simulink model "FSI09_2"  (R2024b)
settings: Solver=FixedStepAuto  StartTime=0.0  StopTime=t_stop  FixedStep=Ts  RelTol=1e-3
values from neighbouring files (symbols this model uses):
  A = 1+exp(-delta*t)    [FSI04WS.m]    (also in FSI09WS.m = [0 1;-k/m -b/m])
  B = [0;1/m]    [FSI09WS.m]
  C = 0.01    [FSI03WS.m]    (also in FSI09WS.m = [1 0])
  D = [0]    [FSI09WS.m]
  F = 1    [FSI08WS.m]    (also in FSI09WS.m = 10)
  f = chirp_end:(chirp_start/(length(t)-1)):chirp_start    [FSI04WS.m]    (also in FSI08WS.m = 5; FSI09WS.m = 5)
  swich = -1    [FSI08WS.m]    (also in FSI09WS.m; FSI10WS.m)
  t_stop = 500    [FSI04WS.m]    (also in FSI07WS.m = 1; FSI08WS.m = 100; FSI09WS.m = 600; FSI10WS.m = 1)
  v0 = 25    [FSI01WS.m]    (also in FSI08WS.m = 0; FSI09WS.m = 0)
  x0 = 1    [FSI04WS.m]    (also in FSI08WS.m = 0; FSI09WS.m = 0)
undefined symbols (not defined in the file or in its folder): den, num
libraries: simulink x1
settings Model: Creator=fmiro  LastModifiedBy=fmiro

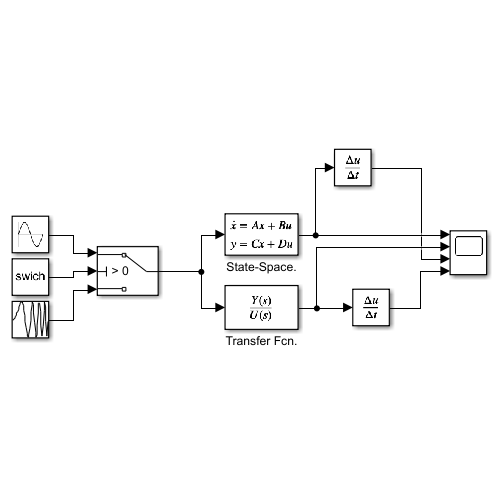
[thumbnail: Simulink's stored preview of the top-level diagram]
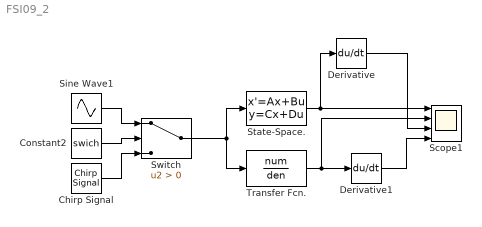
== system FSI09_2 ==
  Chirp Signal : simulink/Sources/Chirp Signal  f1=0  T=t_stop  f2=20
  Constant2 : Constant  Value=swich
  Derivative : Derivative
  Derivative1 : Derivative
  Scope1 : Scope  NumInputPorts=4
  Sine Wave1 : Sin  Amplitude=F  Frequency=2*pi*f  SampleTime=0
  State-Space. : StateSpace  A=A  B=B  C=C  D=D  InitialCondition=[x0 v0]
  Switch : Switch  Criteria=u2 > Threshold  SaturateOnIntegerOverflow=off  InputSameDT=off
  Transfer Fcn. : TransferFcn  Numerator=num  Denominator=den
  wires:
  Switch/1 -> Transfer Fcn./1, State-Space./1
  Transfer Fcn./1 -> Derivative1/1, Scope1/2
  State-Space./1 -> Scope1/1, Derivative/1
  Chirp Signal/1 -> Switch/3
  Sine Wave1/1 -> Switch/1
  Constant2/1 -> Switch/2
  Derivative/1 -> Scope1/3
  Derivative1/1 -> Scope1/4
